simulink model "ex2"  (R2025b)
settings: Solver=VariableStepAuto  StartTime=0.0  StopTime=1  FixedStep=1e-4  RelTol=1e-5
values from neighbouring files (symbols this model uses):
  al = ap * 10    [sim4.m]
  b_a = 2*K^2*(as*J-b)/(3*np^2*psi_nominal)    [sim4.m]
  I_base = sqrt(2) * K * I_n    [sim4.m]
  Id_ref = psi_nominal_pu*psi_base/L_M    [sim4.m]
  ki = ac*(R_s+R_R+R_a)    [sim4.m]
  kis = 2*K^2*as^2*J/(3*np^2*psi_nominal)    [sim4.m]
  kp = ac*L_sig    [sim4.m]
  kps = 2*K^2*as*J/(3*np^2*psi_nominal)    [sim4.m]
  L_M_est = L_M    (= 0.3354)    [sim4.m]
  L_sig = 0.0416    [sim4.m]
  lambda = 1.5    [sim4.m]
  R_a = ac*L_sig -(R_s+R_R)    [sim4.m]
  R_R_est = 2 * R_R    (= 4.212)    [sim4.m]
  R_s = 6.5746    [sim4.m]
  V_base = sqrt(2) * K * V_n    [sim4.m]
  w_base = 2*pi*f_base    (= 314.159265359)    [sim4.m]
  w_delta = 0.1 * w_base    (= 31.4159265359)    [sim4.m]
settings Model: Creator=Dimitris  LastModifiedBy=Dimitris

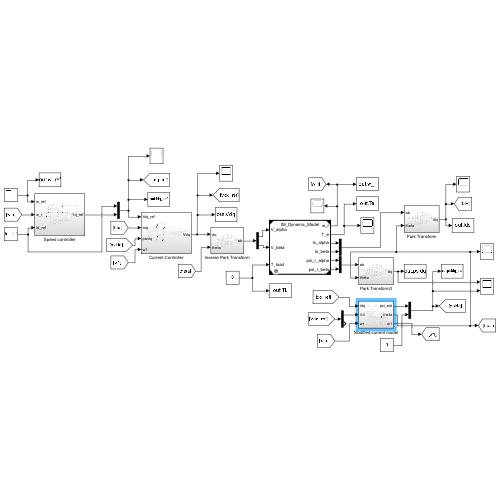
[thumbnail: Simulink's stored preview of the top-level diagram]
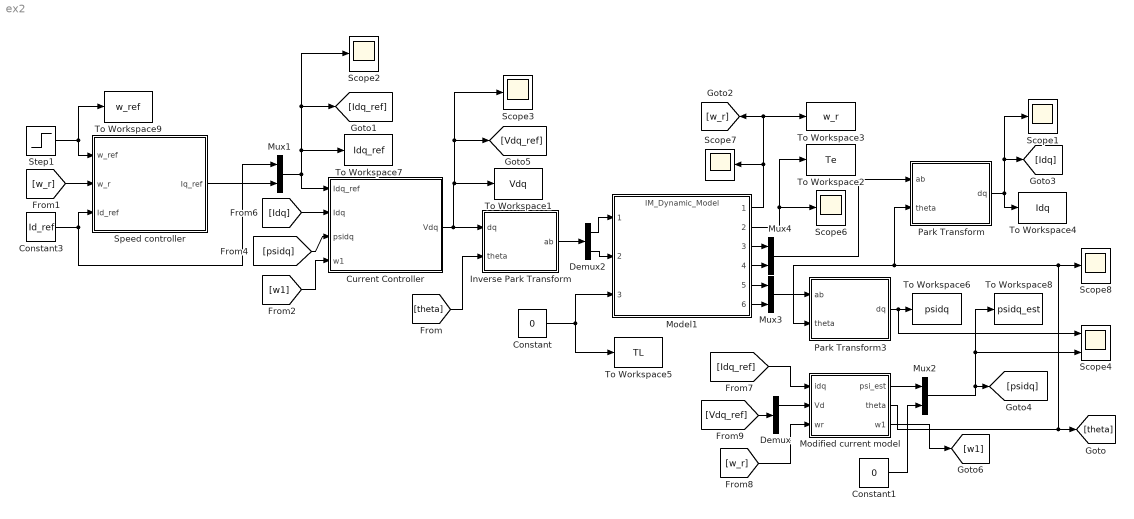
== system ex2 ==
  Constant : Constant  Value=0
  Constant1 : Constant  Value=0
  Constant3 : Constant  Value=Id_ref
  Current Controller : Subsystem
  Demux : Demux  Outputs=2
  Demux2 : Demux  Outputs=2
  Inverse Park Transform : Subsystem
  Model1 : ModelReference  ModelNameDialog=IM_Dynamic_Model.slxp  ModelReferenceVersion=1.0  CopyOfModelProtected=on
  Modified current model : Subsystem
  Mux{1..4} (4 alike) : Mux  Inputs=2
  Park Transform : Subsystem
  Park Transform3 : Subsystem
  Scope{1..3,6..8} (6 alike) : Scope
      Scope1 settings: ActiveDisplayYMinimum=-8.220891656114091  ActiveDisplayYMaximum=8.3565214945093338
      Scope2 settings: ActiveDisplayYMinimum=-5.39157834293709  ActiveDisplayYMaximum=5.39157834293709  DataLoggingVariableName=ScopeData2
      Scope3 settings: ActiveDisplayYMinimum=-84.671660801278563  ActiveDisplayYMaximum=370.537762179255  DataLoggingVariableName=ScopeData3
      Scope6 settings: ActiveDisplayYMinimum=-19.140026431999182  ActiveDisplayYMaximum=45.57557076011858
      Scope7 settings: ActiveDisplayYMinimum=-66.240786944568924  ActiveDisplayYMaximum=468.27046477470873  DataLoggingVariableName=ScopeData6
      Scope8 settings: ActiveDisplayYMinimum=-0.5997953392009252  ActiveDisplayYMaximum=7.0273783123126936  DataLoggingVariableName=ScopeData7
  Scope4 : Scope  NumInputPorts=2
      settings: ActiveDisplayYMinimum=-0.16702830631814142  ActiveDisplayYMaximum=1.4967561233883415  DataLoggingVariableName=ScopeData4
  Speed controller : Subsystem
  Step1 : Step  Time=0.5  Before=1*w_base  After=0.5*w_base  SampleTime=0
  To Workspace1 : ToWorkspace  VariableName=Vdq  SaveFormat=Timeseries  SampleTime=-1
  To Workspace2 : ToWorkspace  VariableName=Te  SaveFormat=Timeseries  SampleTime=-1
  To Workspace3 : ToWorkspace  VariableName=w_r  SaveFormat=Timeseries  SampleTime=-1
  To Workspace4 : ToWorkspace  VariableName=Idq  SaveFormat=Timeseries  SampleTime=-1
  To Workspace5 : ToWorkspace  VariableName=TL  SaveFormat=Timeseries  SampleTime=-1
  To Workspace6 : ToWorkspace  VariableName=psidq  SaveFormat=Timeseries  SampleTime=-1
  To Workspace7 : ToWorkspace  VariableName=Idq_ref  SaveFormat=Timeseries  SampleTime=-1
  To Workspace8 : ToWorkspace  VariableName=psidq_est  SaveFormat=Timeseries  SampleTime=-1
  To Workspace9 : ToWorkspace  VariableName=w_ref  SaveFormat=Timeseries  SampleTime=-1
  wires:
  Current Controller/1(Vdq) -> Scope3/1, [Vdq_ref], To Workspace1/1, Inverse Park Transform/1(dq)
  Mux1/1 -> To Workspace7/1, Scope2/1, [Idq_ref], Current Controller/1(Idq_ref)
  Inverse Park Transform/1(ab) -> Demux2/1
  Model1/4 -> Mux4/2
  Mux4/1 -> Park Transform/1(ab)
  Demux2/1 -> Model1/1
  Park Transform/1(dq) -> To Workspace4/1, [Idq], Scope1/1
  Constant/1 -> To Workspace5/1, Model1/3
  Mux3/1 -> Park Transform3/1(ab)
  Demux2/2 -> Model1/2
  Model1/3 -> Mux4/1
  Model1/2 -> To Workspace2/1, Scope6/1
  Model1/6 -> Mux3/2
  Park Transform3/1(dq) -> Scope4/1, To Workspace6/1
  Model1/1 -> [w_r], To Workspace3/1, Scope7/1
  Model1/5 -> Mux3/1
  [theta] -> Inverse Park Transform/2(theta)
  [psidq] -> Current Controller/3(psidq)
  [w1] -> Current Controller/4(w1)
  Speed controller/1(Iq_ref) -> Mux1/2
  Constant3/1 -> Speed controller/3(Id_ref), Mux1/1
  [w_r] -> Speed controller/2(w_r)
  Step1/1 -> To Workspace9/1, Speed controller/1(w_ref)
  [Idq] -> Current Controller/2(Idq)
  [Idq_ref] -> Modified current model/1(idq)
  [w_r] -> Modified current model/3(wr)
  Modified current model/1(psi_est) -> Mux2/1
  Constant1/1 -> Mux2/2
  Modified current model/2(theta) -> Park Transform3/2(theta), Park Transform/2(theta), Scope8/1, [theta]
  Mux2/1 -> [psidq], Scope4/2, To Workspace8/1
  [Vdq_ref] -> Demux/1
  Demux/1 -> Modified current model/2(Vd)
  Modified current model/3(w1) -> [w1]

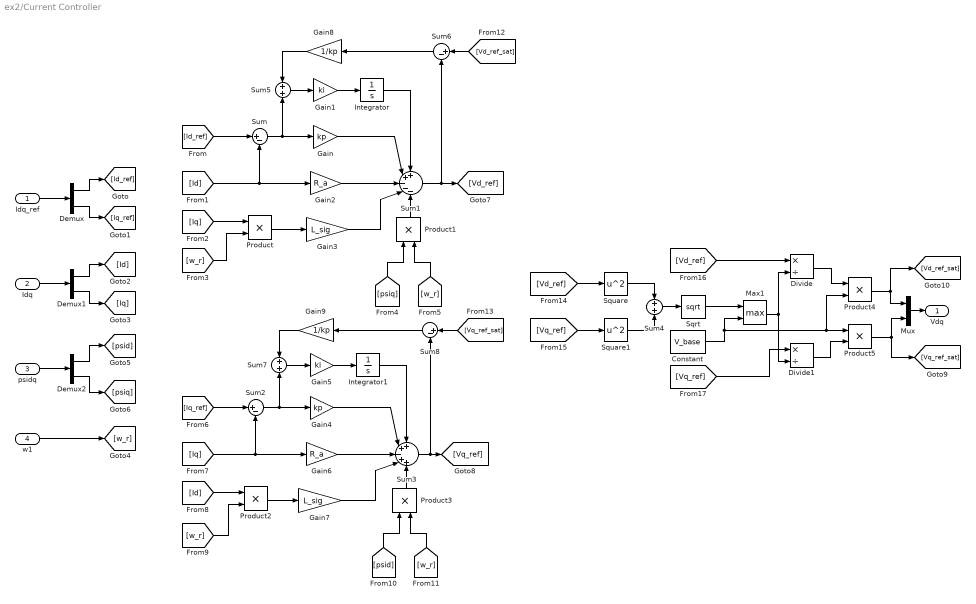
== system ex2/Current Controller ==
  Idq_ref : Inport
  Idq : Inport  Port=2
  psidq : Inport  Port=3
  w1 : Inport  Port=4
  Constant : Constant  Value=V_base
  Demux : Demux  Outputs=2
  Demux1 : Demux  Outputs=2
  Demux2 : Demux  Outputs=2
  Divide : Product  Inputs=*/
  Divide1 : Product  Inputs=*/
  Gain : Gain  Gain=kp
  Gain1 : Gain  Gain=ki
  Gain2 : Gain  Gain=R_a
  Gain3 : Gain  Gain=L_sig
  Gain4 : Gain  Gain=kp
  Gain5 : Gain  Gain=ki
  Gain6 : Gain  Gain=R_a
  Gain7 : Gain  Gain=L_sig
  Gain8 : Gain  Gain=1/kp
  Gain9 : Gain  Gain=1/kp
  Integrator : Integrator
  Integrator1 : Integrator
  Max1 : MinMax  Function=max  Inputs=2
  Mux : Mux  Inputs=2
  Product{,1..5} (6 alike) : Product
  Sqrt : Sqrt
  Square : Math  Operator=square
  Square1 : Math  Operator=square
  Sum{,2,6,8} (4 alike) : Sum  Inputs=|+-
  Sum1 : Sum  Inputs=++---
  Sum3 : Sum  Inputs=++-++
  Sum4 : Sum
  Sum5 : Sum
  Sum7 : Sum
  Vdq : Outport
  wires:
  Idq_ref/1 -> Demux/1
  Idq/1 -> Demux1/1
  Demux/1 -> [Id_ref]
  Demux/2 -> [Iq_ref]
  Demux1/1 -> [Id]
  Demux1/2 -> [Iq]
  [Id_ref] -> Sum/1
  [Id] -> Sum/2, Gain2/1
  Sum/1 -> Sum5/2, Gain/1
  Gain1/1 -> Integrator/1
  Integrator/1 -> Sum1/1
  Gain/1 -> Sum1/2
  Gain2/1 -> Sum1/3
  Gain3/1 -> Sum1/4
  Product/1 -> Gain3/1
  w1/1 -> [w_r]
  [Iq] -> Product/1
  [w_r] -> Product/2
  psidq/1 -> Demux2/1
  Demux2/1 -> [psid]
  Demux2/2 -> [psiq]
  [psiq] -> Product1/1
  [w_r] -> Product1/2
  Product1/1 -> Sum1/5
  Product3/1 -> Sum3/5
  [w_r] -> Product3/2
  [psid] -> Product3/1
  Product2/1 -> Gain7/1
  [Id] -> Product2/1
  Integrator1/1 -> Sum3/1
  Gain6/1 -> Sum3/3
  Gain5/1 -> Integrator1/1
  Gain7/1 -> Sum3/4
  Sum2/1 -> Sum7/2, Gain4/1
  [Iq_ref] -> Sum2/1
  [w_r] -> Product2/2
  [Iq] -> Sum2/2, Gain6/1
  Gain4/1 -> Sum3/2
  Sum1/1 -> [Vd_ref], Sum6/2
  [Vd_ref] -> Square/1
  [Vq_ref] -> Square1/1
  Square/1 -> Sum4/1
  Square1/1 -> Sum4/2
  Sum4/1 -> Sqrt/1
  Sqrt/1 -> Max1/1
  Max1/1 -> Divide/2, Divide1/2
  [Vd_ref] -> Divide/1
  [Vq_ref] -> Divide1/1
  Constant/1 -> Product4/2, Product5/1, Max1/2
  Mux/1 -> Vdq/1
  Sum5/1 -> Gain1/1
  Sum6/1 -> Gain8/1
  [Vd_ref_sat] -> Sum6/1
  Gain8/1 -> Sum5/1
  Sum7/1 -> Gain5/1
  Gain9/1 -> Sum7/1
  Sum3/1 -> Sum8/2, [Vq_ref]
  Sum8/1 -> Gain9/1
  [Vq_ref_sat] -> Sum8/1
  Divide/1 -> Product4/1
  Divide1/1 -> Product5/2
  Product5/1 -> [Vq_ref_sat], Mux/2
  Product4/1 -> [Vd_ref_sat], Mux/1

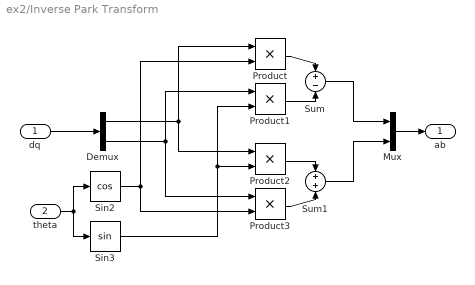
== system ex2/Inverse Park Transform ==
  dq : Inport
  theta : Inport  Port=2
  Demux : Demux  Outputs=2
  Mux : Mux  Inputs=2
  Product{,1..3} (4 alike) : Product
  Sin2 : Trigonometry  Operator=cos
  Sin3 : Trigonometry
  Sum : Sum  Inputs=+-
  Sum1 : Sum
  ab : Outport
  wires:
  Sum1/1 -> Mux/2
  Sin3/1 -> Product2/2, Product1/2
  Product1/1 -> Sum/2
  Demux/1 -> Product2/1, Product/1
  Mux/1 -> ab/1
  dq/1 -> Demux/1
  Sin2/1 -> Product/2, Product3/2
  Demux/2 -> Product1/1, Product3/1
  theta/1 -> Sin3/1, Sin2/1
  Sum/1 -> Mux/1
  Product/1 -> Sum/1
  Product3/1 -> Sum1/2
  Product2/1 -> Sum1/1

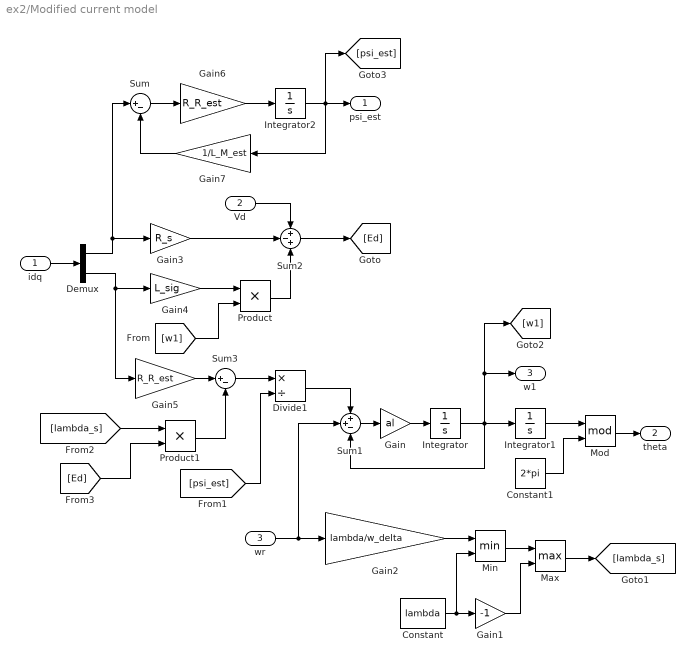
== system ex2/Modified current model ==
  idq : Inport
  Vd : Inport  Port=2
  wr : Inport  Port=3
  Constant : Constant  Value=lambda
  Constant1 : Constant  Value=2*pi
  Demux : Demux  Outputs=2
  Divide1 : Product  Inputs=*/
  Gain : Gain  Gain=al
  Gain1 : Gain  Gain=-1
  Gain2 : Gain  Gain=lambda/w_delta
  Gain3 : Gain  Gain=R_s
  Gain4 : Gain  Gain=L_sig
  Gain5 : Gain  Gain=R_R_est
  Gain6 : Gain  Gain=R_R_est
  Gain7 : Gain  Gain=1/L_M_est
  Integrator : Integrator
  Integrator1 : Integrator
  Integrator2 : Integrator  InitialCondition=0.001
  Max : MinMax  Function=max  Inputs=2
  Min : MinMax  Inputs=2
  Mod : Math  Operator=mod
  Product : Product
  Product1 : Product
  Sum : Sum  Inputs=|+-
  Sum1 : Sum  Inputs=++-
  Sum2 : Sum  Inputs=+-+
  Sum3 : Sum  Inputs=|+-
  psi_est : Outport
  theta : Outport  Port=2
  w1 : Outport  Port=3
  wires:
  idq/1 -> Demux/1
  Constant1/1 -> Mod/2
  Integrator1/1 -> Mod/1
  Mod/1 -> theta/1
  Integrator/1 -> Sum1/3, Integrator1/1, w1/1, [w1]
  Sum2/1 -> [Ed]
  Vd/1 -> Sum2/1
  Gain3/1 -> Sum2/2
  Demux/1 -> Gain3/1, Sum/1
  Demux/2 -> Gain5/1, Gain4/1
  Gain4/1 -> Product/1
  Product/1 -> Sum2/3
  Min/1 -> Max/1
  Gain1/1 -> Max/2
  Constant/1 -> Min/2, Gain1/1
  wr/1 -> Sum1/2, Gain2/1
  Gain2/1 -> Min/1
  Max/1 -> [lambda_s]
  [w1] -> Product/2
  Gain/1 -> Integrator/1
  Sum1/1 -> Gain/1
  Sum3/1 -> Divide1/1
  [psi_est] -> Divide1/2
  Gain5/1 -> Sum3/1
  Product1/1 -> Sum3/2
  [lambda_s] -> Product1/1
  [Ed] -> Product1/2
  Integrator2/1 -> Gain7/1, [psi_est], psi_est/1
  Gain6/1 -> Integrator2/1
  Sum/1 -> Gain6/1
  Gain7/1 -> Sum/2
  Divide1/1 -> Sum1/1

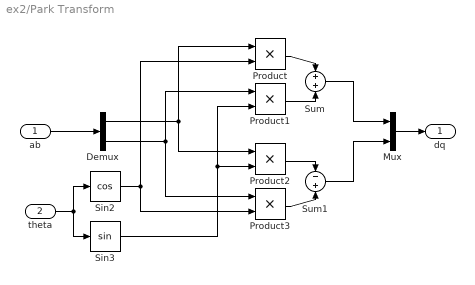
== system ex2/Park Transform ==
  ab : Inport
  theta : Inport  Port=2
  Demux : Demux  Outputs=2
  Mux : Mux  Inputs=2
  Product{,1..3} (4 alike) : Product
  Sin2 : Trigonometry  Operator=cos
  Sin3 : Trigonometry
  Sum : Sum
  Sum1 : Sum  Inputs=-+
  dq : Outport
  wires:
  Sin3/1 -> Product1/2, Product2/2
  Sin2/1 -> Product/2, Product3/2
  theta/1 -> Sin3/1, Sin2/1
  Demux/2 -> Product1/1, Product3/1
  Sum1/1 -> Mux/2
  Sum/1 -> Mux/1
  Demux/1 -> Product2/1, Product/1
  Product2/1 -> Sum1/1
  Product3/1 -> Sum1/2
  Product1/1 -> Sum/2
  Product/1 -> Sum/1
  Mux/1 -> dq/1
  ab/1 -> Demux/1

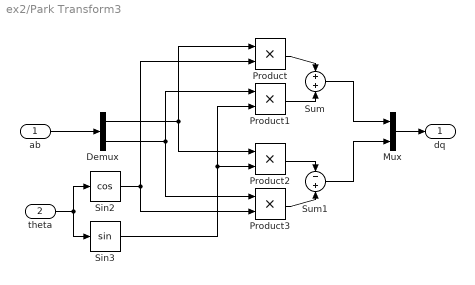
== system ex2/Park Transform3 ==
  ab : Inport
  theta : Inport  Port=2
  Demux : Demux  Outputs=2
  Mux : Mux  Inputs=2
  Product{,1..3} (4 alike) : Product
  Sin2 : Trigonometry  Operator=cos
  Sin3 : Trigonometry
  Sum : Sum
  Sum1 : Sum  Inputs=-+
  dq : Outport
  wires:
  Sin3/1 -> Product1/2, Product2/2
  Sin2/1 -> Product/2, Product3/2
  theta/1 -> Sin3/1, Sin2/1
  Demux/2 -> Product1/1, Product3/1
  Sum1/1 -> Mux/2
  Sum/1 -> Mux/1
  Demux/1 -> Product2/1, Product/1
  Product2/1 -> Sum1/1
  Product3/1 -> Sum1/2
  Product1/1 -> Sum/2
  Product/1 -> Sum/1
  Mux/1 -> dq/1
  ab/1 -> Demux/1

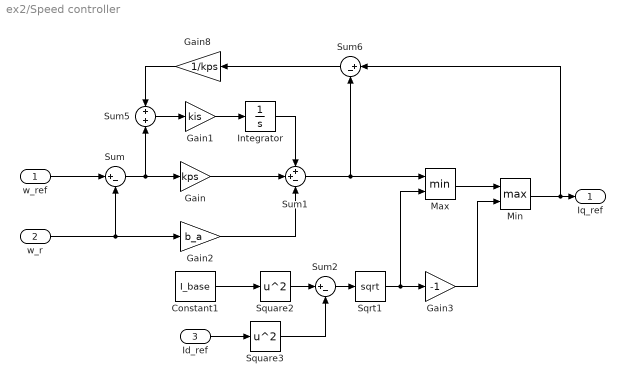
== system ex2/Speed controller ==
  w_ref : Inport
  w_r : Inport  Port=2
  Id_ref : Inport  Port=3
  Constant1 : Constant  Value=I_base
  Gain : Gain  Gain=kps
  Gain1 : Gain  Gain=kis
  Gain2 : Gain  Gain=b_a
  Gain3 : Gain  Gain=-1
  Gain8 : Gain  Gain=1/kps
  Integrator : Integrator
  Max : MinMax  Inputs=2
  Min : MinMax  Function=max  Inputs=2
  Sqrt1 : Sqrt
  Square2 : Math  Operator=square
  Square3 : Math  Operator=square
  Sum : Sum  Inputs=|+-
  Sum1 : Sum  Inputs=++-
  Sum2 : Sum  Inputs=|+-
  Sum5 : Sum
  Sum6 : Sum  Inputs=|+-
  Iq_ref : Outport
  wires:
  w_ref/1 -> Sum/1
  w_r/1 -> Sum/2, Gain2/1
  Sum/1 -> Sum5/2, Gain/1
  Gain1/1 -> Integrator/1
  Integrator/1 -> Sum1/1
  Gain/1 -> Sum1/2
  Gain2/1 -> Sum1/3
  Sum1/1 -> Sum6/2, Max/1
  Sum5/1 -> Gain1/1
  Sum6/1 -> Gain8/1
  Gain8/1 -> Sum5/1
  Sqrt1/1 -> Max/2, Gain3/1
  Sum2/1 -> Sqrt1/1
  Constant1/1 -> Square2/1
  Square2/1 -> Sum2/1
  Id_ref/1 -> Square3/1
  Square3/1 -> Sum2/2
  Max/1 -> Min/1
  Gain3/1 -> Min/2
  Min/1 -> Sum6/1, Iq_ref/1
